simulink library "Wind_Lib"  (R2025a)
settings: Solver=ode45  StartTime=0.0  StopTime=10.0  RelTol=1e-3  EnableMultiTasking=on
undefined symbols (not defined in the file): WT_Params
libraries: nesl_utility x15, sm_lib x9, fl_lib x9, AerodynamicLoads_lib x1, $bdroot x1
Description:
  | Copyright 2009-2025 The MathWorks, Inc.
settings Model: Creator=smiller  LastModifiedBy=smiller
settings SolverCC: AlgebraicLoopSolver=TrustRegion
settings DataIOCC: LimitDataPoints=on  SaveFormat=Array  SignalLoggingSaveFormat=ModelDataLogs  ReturnWorkspaceOutputs=off
settings OptimizationCC: ReuseModelBlockBuffer=off  ExpressionDepthLimit=2147483647.0  LifeSpan=inf
settings DebuggingCC: UnderspecifiedInitializationDetection=Classic  MergeDetectMultiDrivingBlocksExec=none  SolverPrmCheckMsg=warning  FcnCallInpInsideContextMsg=warning  UnconnectedInputMsg=warning  UnconnectedOutputMsg=warning  UnconnectedLineMsg=warning  AllowSymbolicDim=off  StateNameClashWarn=warning  PregeneratedLibrarySubsystemCodeDiagnostic=none  SFUnexpectedBacktrackingDiag=warning  SFNoUnconditionalDefaultTransitionDiag=warning  SFExecutionAtInitializationDiag=none  ArithmeticOperatorsInVariantConditions=warning
settings HardwareCC: ProdBitPerPointer=32.0  ProdBitPerSizeT=32.0  ProdBitPerPtrDiffT=32.0  ProdLargestAtomicFloat=None  ProdIntDivRoundTo=Undefined  ProdEndianess=Unspecified  ProdWordSize=32.0  ProdHWDeviceType=32-bit Generic
settings ModelReferenceCC: EnableRefExpFcnMdlSchedulingChecks=on  PropagateSignalLabelsOutOfModel=off
settings SFSimCC: SimUseLocalCustomCode=off  CustomCodeUndefinedFunction=UseInterfaceOnly
settings RTWCC: RTWUseLocalCustomCode=off  GPUComputeCapability=3.5  DLArmComputeVersion=19.05
settings CodeAppCC: StateflowObjectComments=on
settings GRTTargetCC: TargetLangStandard=C89/C90 (ANSI)  CombineOutputUpdateFcns=off  GRTInterface=on
settings ConfigComp: CovMetricSettings=dw  CovSaveCumulativeToWorkspaceVar=on  CovSaveSingleToWorkspaceVar=on  CovExternalEMLEnable=off  CovSFcnEnable=off

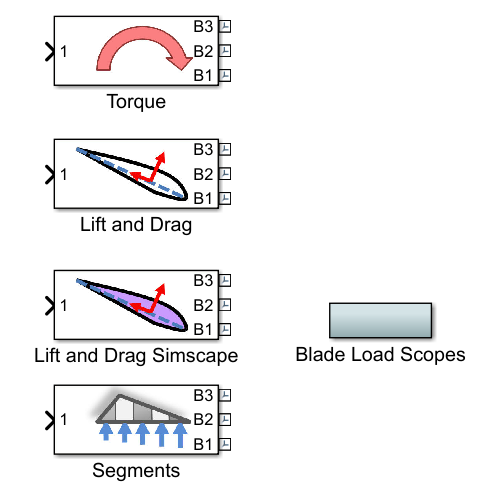
[thumbnail: Simulink's stored preview of the top-level diagram]
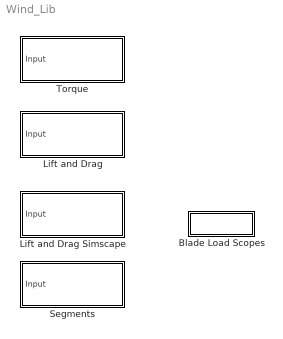
== system Wind_Lib ==
  Blade Load Scopes : Subsystem
  Lift and Drag : Subsystem
      mask Display: image('Blade_Load_Lift_Drag_IMAGE.jpg');
  Lift and Drag Simscape : Subsystem  VariantControl=Lift_and_Drag_Simscape
      mask Display: image('Blade_Load_Lift_Drag_SSC_IMAGE.jpg');
  Segments : Subsystem
      mask Display: image('Blade_Load_Segments_IMAGE.jpg');
  Torque : Subsystem
      mask Display: image('Blade_Load_Torque_IMAGE.jpg');

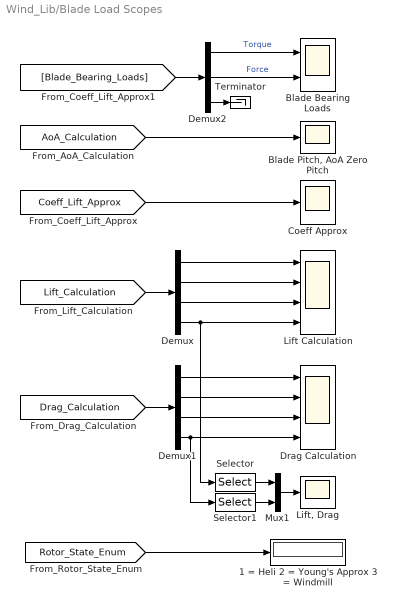
== system Wind_Lib/Blade Load Scopes ==
  1 = Heli 2 = Young's Approx 3 = Windmill : Display
  Blade Bearing Loads : Scope  NumInputPorts=2
      settings: TimeSpan=80  ActiveDisplayYMinimum=-2.0E+6  ActiveDisplayYMaximum=4.0E+6  DataLoggingVariableName=ScopeData10
  "Blade Pitch, AoA Zero Pitch" : Scope
      settings: TimeSpan=400  ActiveDisplayYMinimum=0  ActiveDisplayYMaximum=100  DataLoggingVariableName=ScopeData3
  Coeff Approx : Scope
      settings: TimeSpan=400  ActiveDisplayYMinimum=-0.1139986551164904  ActiveDisplayYMaximum=0.01794057021302797  DataLoggingVariableName=ScopeData4
  Demux : Demux  Outputs=[1 3 3 3]
  Demux1 : Demux  Outputs=[1 3 3 3]
  Demux2 : Demux  Outputs=[3 3 12]
  Drag Calculation : Scope  NumInputPorts=4
      settings: TimeSpan=400  ActiveDisplayYMinimum=-2000  ActiveDisplayYMaximum=4000  DataLoggingVariableName=ScopeData5
  Lift Calculation : Scope  NumInputPorts=4
      settings: TimeSpan=400  ActiveDisplayYMinimum=0  ActiveDisplayYMaximum=2000  DataLoggingVariableName=ScopeData2
  "Lift, Drag" : Scope
      settings: TimeSpan=160  ActiveDisplayYMinimum=-250.43517596694389  ActiveDisplayYMaximum=408.30262213523071
  Mux1 : Mux  Inputs=2
  Selector : Selector  InputPortWidth=3  IndexOptions=Index vector (dialog)  Indices=[1]  OutputSizes=1
  Selector1 : Selector  InputPortWidth=3  IndexOptions=Index vector (dialog)  Indices=[1 3]  OutputSizes=1
  Terminator : Terminator
  wires:
  Demux2/2 -> Blade Bearing Loads/2  "Force"
  Demux2/1 -> Blade Bearing Loads/1  "Torque"
  [Blade_Bearing_Loads] -> Demux2/1
  Selector1/1 -> Mux1/2
  Selector/1 -> Mux1/1
  [AoA_Calculation] -> "Blade Pitch, AoA Zero Pitch"/1
  Mux1/1 -> "Lift, Drag"/1
  [Lift_Calculation] -> Demux/1
  Demux/1 -> Lift Calculation/1
  Demux/2 -> Lift Calculation/2
  Demux/3 -> Lift Calculation/3
  Demux/4 -> Selector/1, Lift Calculation/4
  [Coeff_Lift_Approx] -> Coeff Approx/1
  [Drag_Calculation] -> Demux1/1
  Demux1/1 -> Drag Calculation/1
  Demux1/2 -> Drag Calculation/2
  Demux1/3 -> Drag Calculation/3
  Demux1/4 -> Selector1/1, Drag Calculation/4
  [Rotor_State_Enum] -> 1 = Heli 2 = Young's Approx 3 = Windmill/1
  Demux2/3 -> Terminator/1

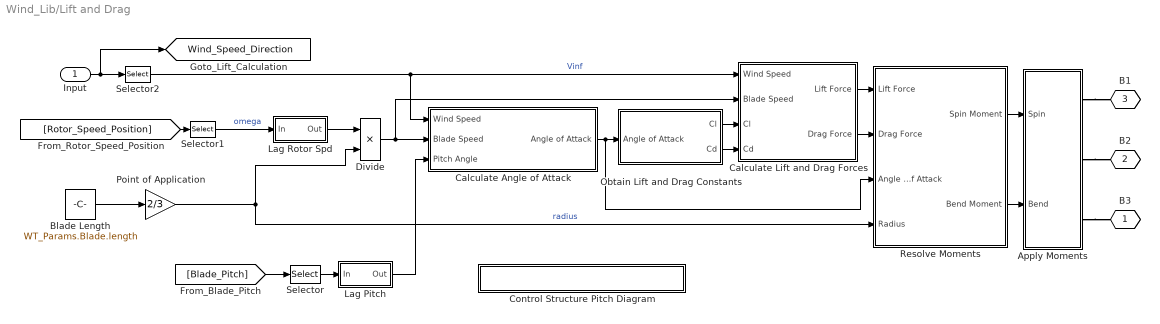
== system Wind_Lib/Lift and Drag ==
  Input : Inport
  Apply Moments : Subsystem
  Blade Length : Constant  Value=WT_Params.Blade.length
  Calculate Angle of Attack : Subsystem
  Calculate Lift and Drag Forces : Subsystem
  Control Structure Pitch Diagram : Subsystem
      mask Display: disp('View Blade Load Diagram');
  Divide : Product  Inputs=**
  Lag Pitch : Subsystem  mask(First-order lag supporting vector signals){b=WT_Params.Lift_Drag_Coeff.time_constant, x_initial=0}
      mask prompts: b "Filter time constant"; x_initial "Initial output"
      mask help: Models a lag of the form 1/(b*s+1) where s is the Laplace operator.
  Lag Rotor Spd : Subsystem  mask(First-order lag supporting vector signals){b=WT_Params.Lift_Drag_Coeff.time_constant, x_initial=0}
      mask prompts: b "Filter time constant"; x_initial "Initial output"
      mask help: Models a lag of the form 1/(b*s+1) where s is the Laplace operator.
  Obtain Lift and Drag Constants : Subsystem
  Point of Application : Gain  Gain=2/3
  Resolve Moments : Subsystem
  Selector : Selector  InputPortWidth=3  IndexOptions=Index vector (dialog)  Indices=[1]  OutputSizes=1
  Selector1 : Selector  InputPortWidth=2  IndexOptions=Index vector (dialog)  Indices=[2]  OutputSizes=1
  Selector2 : Selector  InputPortWidth=2  IndexOptions=Index vector (dialog)  Indices=[1]  OutputSizes=1
  B3 : PMIOPort  Tag=PMCPort  Side=Right
  B2 : PMIOPort  Tag=PMCPort  Port=2  Side=Right
  B1 : PMIOPort  Tag=PMCPort  Port=3  Side=Right
  tag scope: Wind_Speed_Direction=global
  wires:
  Selector/1 -> Lag Pitch/1(In)
  Lag Pitch/1(Out) -> Calculate Angle of Attack/3(Pitch Angle)
  Input/1 -> Selector2/1, [Wind_Speed_Direction]
  Selector2/1 -> Calculate Angle of Attack/1(Wind Speed), Calculate Lift and Drag Forces/1(Wind Speed)  "Vinf"
  Blade Length/1 -> Point of Application/1
  Divide/1 -> Calculate Angle of Attack/2(Blade Speed), Calculate Lift and Drag Forces/2(Blade Speed)
  [Blade_Pitch] -> Selector/1
  Calculate Angle of Attack/1(Angle of Attack) -> Obtain Lift and Drag Constants/1(Angle of Attack), Resolve Moments/3(Angle of Attack)
  Point of Application/1 -> Divide/2, Resolve Moments/4(Radius)  "radius"
  Resolve Moments/2(Bend Moment) -> Apply Moments/2(Bend)
  Resolve Moments/1(Spin Moment) -> Apply Moments/1(Spin)
  [Rotor_Speed_Position] -> Selector1/1
  Selector1/1 -> Lag Rotor Spd/1(In)  "omega"
  Obtain Lift and Drag Constants/1(Cl) -> Calculate Lift and Drag Forces/3(Cl)
  Obtain Lift and Drag Constants/2(Cd) -> Calculate Lift and Drag Forces/4(Cd)
  Calculate Lift and Drag Forces/1(Lift Force) -> Resolve Moments/1(Lift Force)
  Calculate Lift and Drag Forces/2(Drag Force) -> Resolve Moments/2(Drag Force)
  Lag Rotor Spd/1(Out) -> Divide/1
  connections:
  Apply Moments/RConn1 -- B1/RConn1
  Apply Moments/RConn2 -- B2/RConn1
  Apply Moments/RConn3 -- B3/RConn1

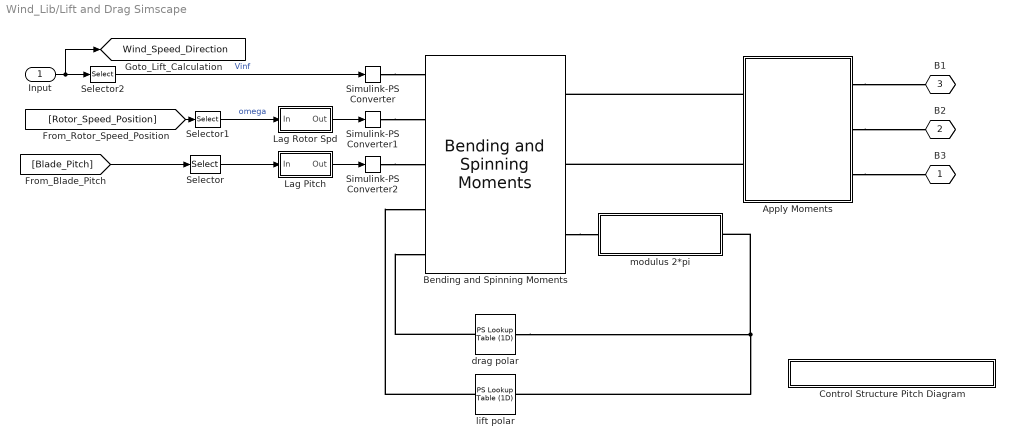
== system Wind_Lib/Lift and Drag Simscape ==
  Input : Inport
  Apply Moments : Subsystem
  Bending and Spinning Moments : AerodynamicLoads_lib/Bending and Spinning Moments  rho=WT_Params.Air.Density kg/m^3  blade_length=WT_Params.Blade.length m  blade_width=WT_Params.Blade.width m  ratio=0.66667  Fl_specify=off  Fl_priority=High  Fl=0 N  Fl_nominal_specify=off  Fl_nominal_value=1  Fl_nominal_unit=N  Fd_specify=off  Fd_priority=High  Fd=0 N  Fd_nominal_specify=off  Fd_nominal_value=1  Fd_nominal_unit=N  v_blade_specify=off  v_blade_priority=High  v_blade=0 m/s  v_blade_nominal_specify=off  v_blade_nominal_value=1  v_blade_nominal_unit=m/s  radius_specify=off  radius_priority=High  radius=0 m  radius_nominal_specify=off  radius_nominal_value=1  radius_nominal_unit=m
      settings: InternalSimscapePortConfiguration="{\"Bottom\":[],\"Left\":[{\"id\":\"v_wind\",\"label\":\"V_wind\",\"type\":\"input\"},{\"id\":\"w_rotor\",\"label\":\"w_rotor\",\"type\":\"input\"},{\"id\":\"theta\",\"label\":\"pitch_angle\",\"type\":\"input\"},{\"id\":\"Cl\",\"label\":\"CL\",\"type\":\"input\"},{\"id\":\"Cd\",\"label\":\"CD\",\"type\":\"input\"}],\"Right\":[{\"id\":\"spin_mom\",\"label\":\"spin\",\"type\":\"output\"},{\"id\":\"bend_mom\",\"label\":\"bend\",\"type\":\"output\"},{\"id\":\"AoA\",\"label\":\"AoA\",\"type\":\"output\"}],\"Top\":[]}"
  Control Structure Pitch Diagram : Subsystem
      mask Display: disp('View Blade Load Diagram');
  Lag Pitch : Subsystem  mask(First-order lag supporting vector signals){b=WT_Params.Lift_Drag_Coeff.time_constant, x_initial=0}
      mask prompts: b "Filter time constant"; x_initial "Initial output"
      mask help: Models a lag of the form 1/(b*s+1) where s is the Laplace operator.
  Lag Rotor Spd : Subsystem  mask(First-order lag supporting vector signals){b=WT_Params.Lift_Drag_Coeff.time_constant, x_initial=0}
      mask prompts: b "Filter time constant"; x_initial "Initial output"
      mask help: Models a lag of the form 1/(b*s+1) where s is the Laplace operator.
  Selector : Selector  InputPortWidth=3  IndexOptions=Index vector (dialog)  Indices=[1]  OutputSizes=1
  Selector1 : Selector  InputPortWidth=2  IndexOptions=Index vector (dialog)  Indices=[2]  OutputSizes=1
  Selector2 : Selector  InputPortWidth=2  IndexOptions=Index vector (dialog)  Indices=[1]  OutputSizes=1
  Simulink-PS Converter : nesl_utility/Simulink-PS Converter  PhysicalDomain=network_engine_domain  SubClassName=ps_input  LeftPortType=input  RightPortType=output  PseudoPeriodic=off  Frequencies=[]  NoiseDistribution=none  NoiseParameters=[]  Unit=m/s  AffineConversion=off  FilteringAndDerivatives=zero  SimscapeFilterOrder=1  InputFilterTimeConstant=0.005  UdotUserProvided=0
  Simulink-PS Converter1 : nesl_utility/Simulink-PS Converter  PhysicalDomain=network_engine_domain  SubClassName=ps_input  LeftPortType=input  RightPortType=output  PseudoPeriodic=off  Frequencies=[]  NoiseDistribution=none  NoiseParameters=[]  Unit=rad/s  AffineConversion=off  FilteringAndDerivatives=zero  SimscapeFilterOrder=1  InputFilterTimeConstant=0.005  UdotUserProvided=0
  Simulink-PS Converter2 : nesl_utility/Simulink-PS Converter  PhysicalDomain=network_engine_domain  SubClassName=ps_input  LeftPortType=input  RightPortType=output  PseudoPeriodic=off  Frequencies=[]  NoiseDistribution=none  NoiseParameters=[]  Unit=rad  AffineConversion=off  FilteringAndDerivatives=zero  SimscapeFilterOrder=1  InputFilterTimeConstant=0.005  UdotUserProvided=0
  drag polar : fl_lib/Physical Signals/Lookup Tables/PS Lookup Table (1D)  x=WT_Params.NACA0015.AoA  f=WT_Params.NACA0015.Cd  interp_method=1  extrap_method=1
  lift polar : fl_lib/Physical Signals/Lookup Tables/PS Lookup Table (1D)  x=WT_Params.NACA0015.AoA  f=WT_Params.NACA0015.Cl  interp_method=1  extrap_method=1
  modulus 2*pi : Subsystem
  B3 : PMIOPort  Tag=PMCPort  Side=Right
  B2 : PMIOPort  Tag=PMCPort  Port=2  Side=Right
  B1 : PMIOPort  Tag=PMCPort  Port=3  Side=Right
  tag scope: Wind_Speed_Direction=global
  wires:
  [Rotor_Speed_Position] -> Selector1/1
  [Blade_Pitch] -> Selector/1
  Input/1 -> [Wind_Speed_Direction], Selector2/1
  Selector2/1 -> Simulink-PS Converter/1  "Vinf"
  Selector1/1 -> Lag Rotor Spd/1(In)  "omega"
  Selector/1 -> Lag Pitch/1(In)
  Lag Rotor Spd/1(Out) -> Simulink-PS Converter1/1
  Lag Pitch/1(Out) -> Simulink-PS Converter2/1
  connections:
  Apply Moments/RConn3 -- B3/RConn1
  Apply Moments/RConn2 -- B2/RConn1
  Apply Moments/RConn1 -- B1/RConn1
  Simulink-PS Converter/RConn1 -- Bending and Spinning Moments/LConn1
  Simulink-PS Converter1/RConn1 -- Bending and Spinning Moments/LConn2
  Simulink-PS Converter2/RConn1 -- Bending and Spinning Moments/LConn3
  Bending and Spinning Moments/RConn3 -- modulus 2*pi/LConn1
  drag polar/LConn1 -- modulus 2*pi/RConn1 -- lift polar/LConn1
  drag polar/RConn1 -- Bending and Spinning Moments/LConn5
  lift polar/RConn1 -- Bending and Spinning Moments/LConn4
  Apply Moments/LConn1 -- Bending and Spinning Moments/RConn1
  Apply Moments/LConn2 -- Bending and Spinning Moments/RConn2

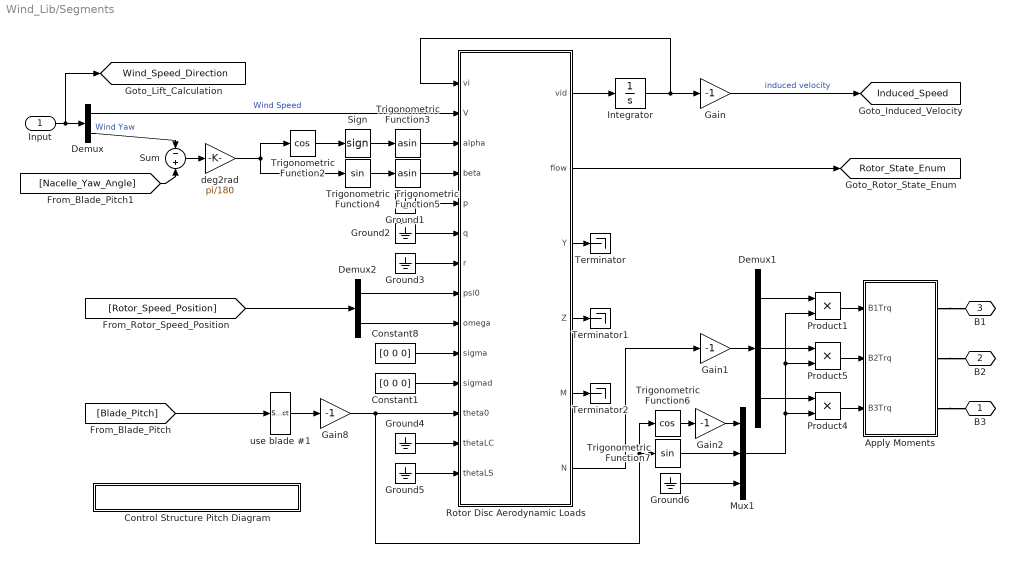
== system Wind_Lib/Segments ==
  Input : Inport
  Apply Moments : Subsystem
  Constant1 : Constant  Value=[0 0 0]
  Constant8 : Constant  Value=[0 0 0]
  Control Structure Pitch Diagram : Subsystem
      mask Display: disp('View Blade Load Diagram');
  Demux : Demux  Outputs=2
  Demux1 : Demux  Outputs=3
  Demux2 : Demux  Outputs=2
  Gain{,1..2,8} (4 alike) : Gain  Gain=-1
  Ground{1..6} (6 alike) : Ground
  Integrator : Integrator
  Mux1 : Mux  Inputs=3
  Product1 : Product  RndMeth=Zero
  Product4 : Product  RndMeth=Zero
  Product5 : Product  RndMeth=Zero
  Rotor Disc Aerodynamic Loads : MATLAB Function  TreatAsAtomicUnit=on  SystemSampleTime=0.01
  Sign : Signum
  Sum : Sum  Inputs=-|+
  Terminator : Terminator
  Terminator1 : Terminator
  Terminator2 : Terminator
  Trigonometric Function2 : Trigonometry  Operator=cos
  Trigonometric Function3 : Trigonometry  Operator=asin
  Trigonometric Function4 : Trigonometry
  Trigonometric Function5 : Trigonometry  Operator=asin
  Trigonometric Function6 : Trigonometry  Operator=cos
  Trigonometric Function7 : Trigonometry
  deg2rad : Gain  Gain=pi/180
  use blade #1 : Selector  InputPortWidth=3  IndexOptions=Index vector (dialog)  Indices=[1]  OutputSizes=1
  B3 : PMIOPort  Side=Right
  B2 : PMIOPort  Port=2  Side=Right
  B1 : PMIOPort  Port=3  Side=Right
  tag scope: Induced_Speed=global, Rotor_State_Enum=global, Wind_Speed_Direction=global
  wires:
  Rotor Disc Aerodynamic Loads/2(flow) -> [Rotor_State_Enum]
  [Rotor_Speed_Position] -> Demux2/1
  [Blade_Pitch] -> use blade #1/1
  Integrator/1 -> Gain/1, Rotor Disc Aerodynamic Loads/1(vi)
  Demux/1 -> Rotor Disc Aerodynamic Loads/2(V)  "Wind Speed"
  Demux/2 -> Sum/1  "Wind Yaw"
  Input/1 -> Demux/1, [Wind_Speed_Direction]
  Gain/1 -> [Induced_Speed]  "induced velocity"
  use blade #1/1 -> Gain8/1
  Gain8/1 -> Rotor Disc Aerodynamic Loads/12(theta0), Trigonometric Function7/1, Trigonometric Function6/1
  Ground1/1 -> Rotor Disc Aerodynamic Loads/5(p)
  Ground2/1 -> Rotor Disc Aerodynamic Loads/6(q)
  Ground3/1 -> Rotor Disc Aerodynamic Loads/7(r)
  Demux2/1 -> Rotor Disc Aerodynamic Loads/8(psi0)
  Demux2/2 -> Rotor Disc Aerodynamic Loads/9(omega)
  Constant8/1 -> Rotor Disc Aerodynamic Loads/10(sigma)
  Constant1/1 -> Rotor Disc Aerodynamic Loads/11(sigmad)
  Ground4/1 -> Rotor Disc Aerodynamic Loads/13(thetaLC)
  Ground5/1 -> Rotor Disc Aerodynamic Loads/14(thetaLS)
  Rotor Disc Aerodynamic Loads/1(vid) -> Integrator/1
  Rotor Disc Aerodynamic Loads/6(N) -> Gain1/1
  Rotor Disc Aerodynamic Loads/3(Y) -> Terminator/1
  Rotor Disc Aerodynamic Loads/4(Z) -> Terminator1/1
  Rotor Disc Aerodynamic Loads/5(M) -> Terminator2/1
  Trigonometric Function2/1 -> Sign/1
  Sign/1 -> Trigonometric Function3/1
  Trigonometric Function3/1 -> Rotor Disc Aerodynamic Loads/3(alpha)
  Trigonometric Function4/1 -> Trigonometric Function5/1
  Trigonometric Function5/1 -> Rotor Disc Aerodynamic Loads/4(beta)
  [Nacelle_Yaw_Angle] -> Sum/2
  Sum/1 -> deg2rad/1
  Ground6/1 -> Mux1/3
  Trigonometric Function7/1 -> Mux1/2
  Trigonometric Function6/1 -> Gain2/1
  Gain1/1 -> Demux1/1
  Demux1/1 -> Product1/1
  Demux1/2 -> Product5/1
  Demux1/3 -> Product4/1
  Mux1/1 -> Product4/2, Product1/2, Product5/2
  deg2rad/1 -> Trigonometric Function2/1, Trigonometric Function4/1
  Gain2/1 -> Mux1/1
  Product1/1 -> Apply Moments/1(B1Trq)
  Product5/1 -> Apply Moments/2(B2Trq)
  Product4/1 -> Apply Moments/3(B3Trq)
  connections:
  Apply Moments/RConn1 -- B1/RConn1
  Apply Moments/RConn2 -- B2/RConn1
  Apply Moments/RConn3 -- B3/RConn1

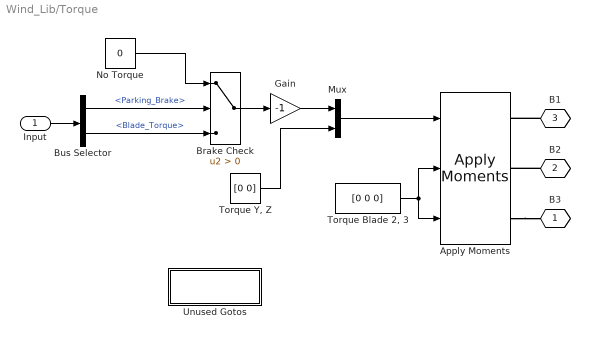
== system Wind_Lib/Torque ==
  Input : Inport
  Apply Moments : $bdroot/Segments/Apply Moments  SystemSampleTime=-1  VariantActivationTime=update diagram  EmptyChoice=off  PassThrough=off  PassThroughVariantControl=(default)  EmptyChoiceVariantControl=(default)  AllowFlexibleInterface=on  Latency=0  AutoFrameSizeCalculation=off
  Brake Check : Switch  Criteria=u2 > Threshold  SaturateOnIntegerOverflow=off  InputSameDT=off
  Bus Selector : BusSelector  OutputSignals=Parking_Brake,Blade_Torque
  Gain : Gain  Gain=-1
  Mux : Mux  Inputs=2
  No Torque : Constant  Value=0
  "Torque Blade 2, 3" : Constant  Value=[0 0 0]
  "Torque Y, Z" : Constant  Value=[0 0]
  Unused Gotos : Subsystem
  B3 : PMIOPort  Tag=PMCPort  Side=Right
  B2 : PMIOPort  Tag=PMCPort  Port=2  Side=Right
  B1 : PMIOPort  Tag=PMCPort  Port=3  Side=Right
  wires:
  Bus Selector/2 -> Brake Check/3  "<Blade_Torque>"
  Bus Selector/1 -> Brake Check/2  "<Parking_Brake>"
  No Torque/1 -> Brake Check/1
  "Torque Blade 2, 3"/1 -> Apply Moments/2, Apply Moments/3
  Mux/1 -> Apply Moments/1
  "Torque Y, Z"/1 -> Mux/2
  Input/1 -> Bus Selector/1
  Brake Check/1 -> Gain/1
  Gain/1 -> Mux/1
  connections:
  B1/RConn1 -- Apply Moments/RConn1
  B2/RConn1 -- Apply Moments/RConn2
  Apply Moments/RConn3 -- B3/RConn1

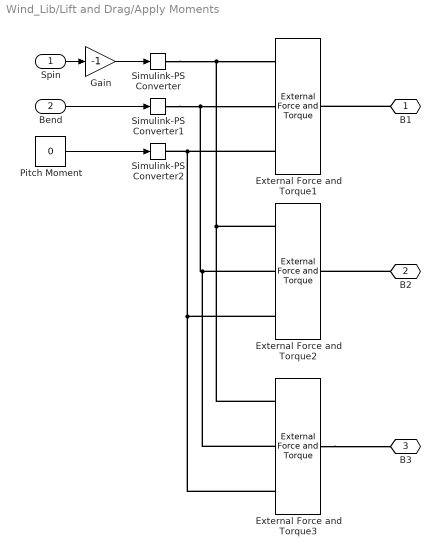
== system Wind_Lib/Lift and Drag/Apply Moments ==
  Spin : Inport
  Bend : Inport  Port=2
  External Force and Torque1 : sm_lib/Forces and Torques/External Force and Torque  EnableForceX=off  EnableForceY=off  EnableForceZ=off  EnableForce=off  ForceResolutionFrame=AttachedFrame  EnableTorqueX=on  EnableTorqueY=on  EnableTorqueZ=on  EnableTorque=off  TorqueResolutionFrame=AttachedFrame
  External Force and Torque2 : sm_lib/Forces and Torques/External Force and Torque  EnableForceX=off  EnableForceY=off  EnableForceZ=off  EnableForce=off  ForceResolutionFrame=AttachedFrame  EnableTorqueX=on  EnableTorqueY=on  EnableTorqueZ=on  EnableTorque=off  TorqueResolutionFrame=AttachedFrame
  External Force and Torque3 : sm_lib/Forces and Torques/External Force and Torque  EnableForceX=off  EnableForceY=off  EnableForceZ=off  EnableForce=off  ForceResolutionFrame=AttachedFrame  EnableTorqueX=on  EnableTorqueY=on  EnableTorqueZ=on  EnableTorque=off  TorqueResolutionFrame=AttachedFrame
  Gain : Gain  Gain=-1
  Pitch Moment : Constant  Value=0
  Simulink-PS Converter : nesl_utility/Simulink-PS Converter  PhysicalDomain=network_engine_domain  SubClassName=ps_input  LeftPortType=input  RightPortType=output  PseudoPeriodic=off  Frequencies=[]  NoiseDistribution=none  NoiseParameters=[]  Unit=1  AffineConversion=off  FilteringAndDerivatives=zero  SimscapeFilterOrder=1  InputFilterTimeConstant=0.005  UdotUserProvided=[]
  Simulink-PS Converter1 : nesl_utility/Simulink-PS Converter  PhysicalDomain=network_engine_domain  SubClassName=ps_input  LeftPortType=input  RightPortType=output  PseudoPeriodic=off  Frequencies=[]  NoiseDistribution=none  NoiseParameters=[]  Unit=1  AffineConversion=off  FilteringAndDerivatives=zero  SimscapeFilterOrder=1  InputFilterTimeConstant=0.005  UdotUserProvided=[]
  Simulink-PS Converter2 : nesl_utility/Simulink-PS Converter  PhysicalDomain=network_engine_domain  SubClassName=ps_input  LeftPortType=input  RightPortType=output  PseudoPeriodic=off  Frequencies=[]  NoiseDistribution=none  NoiseParameters=[]  Unit=1  AffineConversion=off  FilteringAndDerivatives=zero  SimscapeFilterOrder=1  InputFilterTimeConstant=0.005  UdotUserProvided=[]
  B1 : PMIOPort  Side=Right
  B2 : PMIOPort  Port=2  Side=Right
  B3 : PMIOPort  Port=3  Side=Right
  wires:
  Bend/1 -> Simulink-PS Converter1/1
  Gain/1 -> Simulink-PS Converter/1
  Pitch Moment/1 -> Simulink-PS Converter2/1
  Spin/1 -> Gain/1
  connections:
  Simulink-PS Converter/RConn1 -- External Force and Torque3/LConn1 -- External Force and Torque2/LConn1 -- External Force and Torque1/LConn1
  Simulink-PS Converter1/RConn1 -- External Force and Torque3/LConn2 -- External Force and Torque2/LConn2 -- External Force and Torque1/LConn2
  External Force and Torque1/LConn3 -- Simulink-PS Converter2/RConn1 -- External Force and Torque3/LConn3 -- External Force and Torque2/LConn3
  B1/RConn1 -- External Force and Torque1/RConn1
  B2/RConn1 -- External Force and Torque2/RConn1
  External Force and Torque3/RConn1 -- B3/RConn1

== system Wind_Lib/Lift and Drag/Calculate Angle of Attack ==
  Wind Speed : Inport
  Blade Speed : Inport  Port=2
  Pitch Angle : Inport  Port=3
  Subtract : Sum  Inputs=+-
  Trigonometric Function : Trigonometry  Operator=atan2
  Angle of Attack : Outport  VectorParamsAs1DForOutWhenUnconnected=off
  wires:
  Trigonometric Function/1 -> Subtract/1
  Wind Speed/1 -> Trigonometric Function/1
  Blade Speed/1 -> Trigonometric Function/2
  Subtract/1 -> Angle of Attack/1  "alpha"
  Pitch Angle/1 -> Subtract/2  "theta"

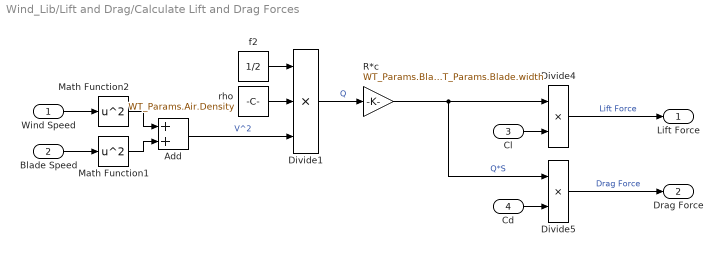
== system Wind_Lib/Lift and Drag/Calculate Lift and Drag Forces ==
  Wind Speed : Inport
  Blade Speed : Inport  Port=2
  Cl : Inport  Port=3
  Cd : Inport  Port=4
  Add : Sum
  Divide1 : Product  Inputs=***
  Divide4 : Product  Inputs=**
  Divide5 : Product  Inputs=**
  Math Function1 : Math  Operator=square  SignedPower=on
  Math Function2 : Math  Operator=square  SignedPower=on
  R*c : Gain  Gain=WT_Params.Blade.length*WT_Params.Blade.width
  f2 : Constant  Value=1/2
  rho : Constant  Value=WT_Params.Air.Density
  Lift Force : Outport  VectorParamsAs1DForOutWhenUnconnected=off
  Drag Force : Outport  Port=2  VectorParamsAs1DForOutWhenUnconnected=off
  wires:
  Math Function2/1 -> Add/1
  Math Function1/1 -> Add/2
  Add/1 -> Divide1/3  "V^2"
  rho/1 -> Divide1/2
  f2/1 -> Divide1/1
  Divide1/1 -> R*c/1  "Q"
  R*c/1 -> Divide4/1, Divide5/1  "Q*S"
  Wind Speed/1 -> Math Function2/1
  Blade Speed/1 -> Math Function1/1
  Divide4/1 -> Lift Force/1  "Lift Force"
  Cl/1 -> Divide4/2
  Divide5/1 -> Drag Force/1  "Drag Force"
  Cd/1 -> Divide5/2

== system Wind_Lib/Lift and Drag/Control Structure Pitch Diagram ==
  Subsystem : Subsystem
      mask Display: image(imread('Blade_Load_Calculation_IMAGE.jpg'));

== system Wind_Lib/Lift and Drag/Lag Pitch ==
  In : Inport
  Gain : Gain  Gain=1/b
  Integrator : Integrator  InitialCondition=x_initial
  Sum : Sum  Inputs=|+-  InputSameDT=on  SaturateOnIntegerOverflow=on  OutDataTypeStr=Inherit: Same as first input
  Out : Outport  VectorParamsAs1DForOutWhenUnconnected=off
  wires:
  Sum/1 -> Integrator/1
  In/1 -> Sum/1
  Integrator/1 -> Gain/1
  Gain/1 -> Sum/2, Out/1

== system Wind_Lib/Lift and Drag/Lag Rotor Spd ==
  In : Inport
  Gain : Gain  Gain=1/b
  Integrator : Integrator  InitialCondition=x_initial
  Sum : Sum  Inputs=|+-  InputSameDT=on  SaturateOnIntegerOverflow=on  OutDataTypeStr=Inherit: Same as first input
  Out : Outport  VectorParamsAs1DForOutWhenUnconnected=off
  wires:
  Gain/1 -> Out/1, Sum/2
  Integrator/1 -> Gain/1
  In/1 -> Sum/1
  Sum/1 -> Integrator/1

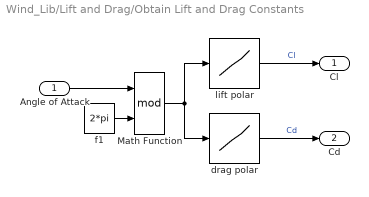
== system Wind_Lib/Lift and Drag/Obtain Lift and Drag Constants ==
  Angle of Attack : Inport
  Math Function : Math  Operator=mod  SignedPower=on
  drag polar : Lookup  InputValues=WT_Params.NACA0015.AoA  Table=WT_Params.NACA0015.Cd  SaturateOnIntegerOverflow=off
  f1 : Constant  Value=2*pi
  lift polar : Lookup  InputValues=WT_Params.NACA0015.AoA  Table=WT_Params.NACA0015.Cl  SaturateOnIntegerOverflow=off
  Cl : Outport  VectorParamsAs1DForOutWhenUnconnected=off
  Cd : Outport  Port=2  VectorParamsAs1DForOutWhenUnconnected=off
  wires:
  f1/1 -> Math Function/2
  Math Function/1 -> lift polar/1, drag polar/1
  Angle of Attack/1 -> Math Function/1
  lift polar/1 -> Cl/1  "Cl"
  drag polar/1 -> Cd/1  "Cd"

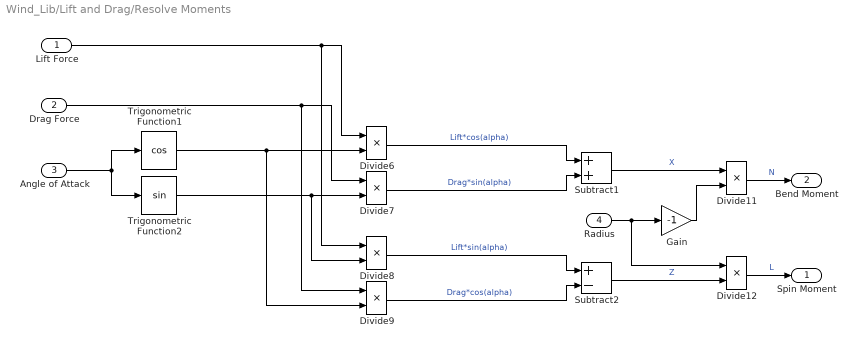
== system Wind_Lib/Lift and Drag/Resolve Moments ==
  Lift Force : Inport
  Drag Force : Inport  Port=2
  Angle of Attack : Inport  Port=3
  Radius : Inport  Port=4
  Divide{6..9,11..12} (6 alike) : Product  Inputs=**
  Gain : Gain  Gain=-1
  Subtract1 : Sum
  Subtract2 : Sum  Inputs=+-
  Trigonometric Function1 : Trigonometry  Operator=cos
  Trigonometric Function2 : Trigonometry
  Spin Moment : Outport  VectorParamsAs1DForOutWhenUnconnected=off
  Bend Moment : Outport  Port=2  VectorParamsAs1DForOutWhenUnconnected=off
  wires:
  Lift Force/1 -> Divide6/1, Divide8/1
  Drag Force/1 -> Divide7/1, Divide9/1
  Trigonometric Function1/1 -> Divide6/2, Divide9/2
  Trigonometric Function2/1 -> Divide7/2, Divide8/2
  Divide6/1 -> Subtract1/1  "Lift*cos(alpha)"
  Divide7/1 -> Subtract1/2  "Drag*sin(alpha)"
  Divide8/1 -> Subtract2/1  "Lift*sin(alpha)"
  Divide9/1 -> Subtract2/2  "Drag*cos(alpha)"
  Subtract1/1 -> Divide11/1  "X"
  Subtract2/1 -> Divide12/2  "Z"
  Gain/1 -> Divide11/2
  Angle of Attack/1 -> Trigonometric Function1/1, Trigonometric Function2/1
  Radius/1 -> Gain/1, Divide12/1
  Divide11/1 -> Bend Moment/1  "N"
  Divide12/1 -> Spin Moment/1  "L"

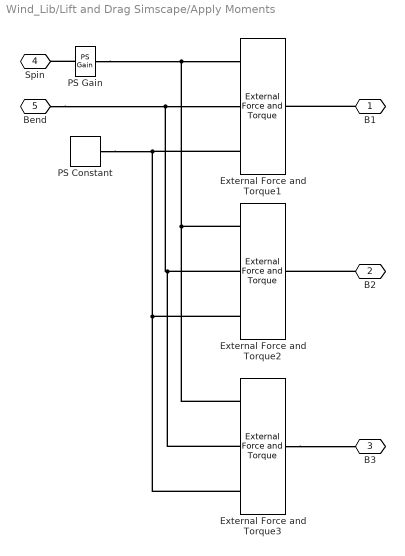
== system Wind_Lib/Lift and Drag Simscape/Apply Moments ==
  External Force and Torque1 : sm_lib/Forces and Torques/External Force and Torque  EnableForceX=off  EnableForceY=off  EnableForceZ=off  EnableForce=off  ForceResolutionFrame=AttachedFrame  EnableTorqueX=on  EnableTorqueY=on  EnableTorqueZ=on  EnableTorque=off  TorqueResolutionFrame=AttachedFrame
  External Force and Torque2 : sm_lib/Forces and Torques/External Force and Torque  EnableForceX=off  EnableForceY=off  EnableForceZ=off  EnableForce=off  ForceResolutionFrame=AttachedFrame  EnableTorqueX=on  EnableTorqueY=on  EnableTorqueZ=on  EnableTorque=off  TorqueResolutionFrame=AttachedFrame
  External Force and Torque3 : sm_lib/Forces and Torques/External Force and Torque  EnableForceX=off  EnableForceY=off  EnableForceZ=off  EnableForce=off  ForceResolutionFrame=AttachedFrame  EnableTorqueX=on  EnableTorqueY=on  EnableTorqueZ=on  EnableTorque=off  TorqueResolutionFrame=AttachedFrame
  PS Constant : fl_lib/Physical Signals/Sources/PS Constant  constant=0
  PS Gain : fl_lib/Physical Signals/Functions/PS Gain  gain=-1
  B1 : PMIOPort  Side=Right
  B2 : PMIOPort  Port=2  Side=Right
  B3 : PMIOPort  Port=3  Side=Right
  Spin : PMIOPort  Port=4  Side=Left
  Bend : PMIOPort  Port=5  Side=Left
  connections:
  External Force and Torque3/LConn1 -- External Force and Torque2/LConn1 -- PS Gain/RConn1 -- External Force and Torque1/LConn1
  External Force and Torque3/LConn2 -- External Force and Torque2/LConn2 -- Bend/RConn1 -- External Force and Torque1/LConn2
  External Force and Torque1/LConn3 -- PS Constant/RConn1 -- External Force and Torque3/LConn3 -- External Force and Torque2/LConn3
  B1/RConn1 -- External Force and Torque1/RConn1
  B2/RConn1 -- External Force and Torque2/RConn1
  External Force and Torque3/RConn1 -- B3/RConn1
  PS Gain/LConn1 -- Spin/RConn1

== system Wind_Lib/Lift and Drag Simscape/Control Structure Pitch Diagram ==
  Subsystem : Subsystem
      mask Display: image(imread('Blade_Load_Calculation_IMAGE.jpg'));

== system Wind_Lib/Lift and Drag Simscape/Lag Pitch ==
  In : Inport
  Gain : Gain  Gain=1/b
  Integrator : Integrator  InitialCondition=x_initial
  Sum : Sum  Inputs=|+-  InputSameDT=on  SaturateOnIntegerOverflow=on  OutDataTypeStr=Inherit: Same as first input
  Out : Outport  VectorParamsAs1DForOutWhenUnconnected=off
  wires:
  Sum/1 -> Integrator/1
  In/1 -> Sum/1
  Integrator/1 -> Gain/1
  Gain/1 -> Sum/2, Out/1

== system Wind_Lib/Lift and Drag Simscape/Lag Rotor Spd ==
  In : Inport
  Gain : Gain  Gain=1/b
  Integrator : Integrator  InitialCondition=x_initial
  Sum : Sum  Inputs=|+-  InputSameDT=on  SaturateOnIntegerOverflow=on  OutDataTypeStr=Inherit: Same as first input
  Out : Outport  VectorParamsAs1DForOutWhenUnconnected=off
  wires:
  Gain/1 -> Out/1, Sum/2
  Integrator/1 -> Gain/1
  In/1 -> Sum/1
  Sum/1 -> Integrator/1

== system Wind_Lib/Lift and Drag Simscape/modulus 2*pi ==
  2*pi : fl_lib/Physical Signals/Sources/PS Constant  constant=2*pi rad
  PS Divide : fl_lib/Physical Signals/Functions/PS Divide
  PS Floor : fl_lib/Physical Signals/Nonlinear Operators/PS Floor
      settings: InternalSimscapePortConfiguration="{\"Bottom\":[],\"Left\":[{\"id\":\"I\",\"label\":\"\",\"type\":\"input\"}],\"Right\":[{\"id\":\"O\",\"label\":\"\",\"type\":\"output\"}],\"Top\":[]}"
  PS Product : fl_lib/Physical Signals/Functions/PS Product
  PS Subtract : fl_lib/Physical Signals/Functions/PS Subtract
  AoA : PMIOPort  Side=Left
  mod(AoA,2*pi) : PMIOPort  Port=2  Side=Right
  connections:
  2*pi/RConn1 -- PS Product/LConn2 -- PS Divide/LConn2
  AoA/RConn1 -- PS Subtract/LConn1 -- PS Divide/LConn1
  PS Divide/RConn1 -- PS Floor/LConn1
  PS Product/LConn1 -- PS Floor/RConn1
  PS Subtract/LConn2 -- PS Product/RConn1
  mod(AoA,2*pi)/RConn1 -- PS Subtract/RConn1

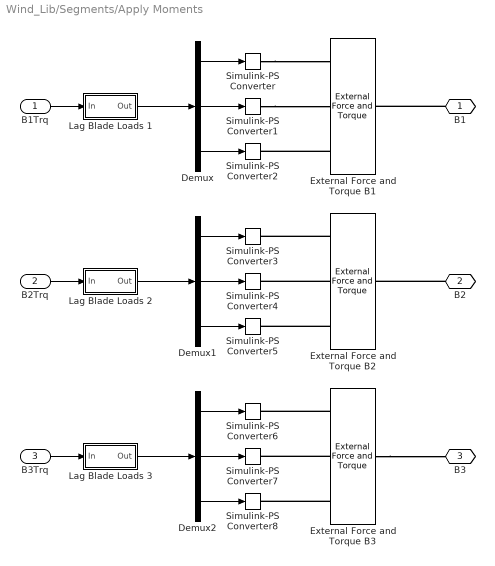
== system Wind_Lib/Segments/Apply Moments ==
  B1Trq : Inport
  B2Trq : Inport  Port=2
  B3Trq : Inport  Port=3
  Demux : Demux  Outputs=3
  Demux1 : Demux  Outputs=3
  Demux2 : Demux  Outputs=3
  External Force and Torque B1 : sm_lib/Forces and Torques/External Force and Torque  EnableForceX=off  EnableForceY=off  EnableForceZ=off  EnableForce=off  ForceResolutionFrame=AttachedFrame  EnableTorqueX=on  EnableTorqueY=on  EnableTorqueZ=on  EnableTorque=off  TorqueResolutionFrame=AttachedFrame
  External Force and Torque B3 : sm_lib/Forces and Torques/External Force and Torque  EnableForceX=off  EnableForceY=off  EnableForceZ=off  EnableForce=off  ForceResolutionFrame=AttachedFrame  EnableTorqueX=on  EnableTorqueY=on  EnableTorqueZ=on  EnableTorque=off  TorqueResolutionFrame=AttachedFrame
  External Force and Torque B2 : sm_lib/Forces and Torques/External Force and Torque  EnableForceX=off  EnableForceY=off  EnableForceZ=off  EnableForce=off  ForceResolutionFrame=AttachedFrame  EnableTorqueX=on  EnableTorqueY=on  EnableTorqueZ=on  EnableTorque=off  TorqueResolutionFrame=AttachedFrame
  Lag Blade Loads 1 : Subsystem  mask(First-order lag supporting vector signals){b=WT_Params.Lift_Drag_Coeff.time_constant, x_initial=0}
      mask prompts: b "Filter time constant"; x_initial "Initial output"
      mask help: Models a lag of the form 1/(b*s+1) where s is the Laplace operator.
  Lag Blade Loads 2 : Subsystem  mask(First-order lag supporting vector signals){b=WT_Params.Lift_Drag_Coeff.time_constant, x_initial=0}
      mask prompts: b "Filter time constant"; x_initial "Initial output"
      mask help: Models a lag of the form 1/(b*s+1) where s is the Laplace operator.
  Lag Blade Loads 3 : Subsystem  mask(First-order lag supporting vector signals){b=WT_Params.Lift_Drag_Coeff.time_constant, x_initial=0}
      mask prompts: b "Filter time constant"; x_initial "Initial output"
      mask help: Models a lag of the form 1/(b*s+1) where s is the Laplace operator.
  Simulink-PS Converter{,1..8} (9 alike) : nesl_utility/Simulink-PS Converter  PhysicalDomain=network_engine_domain  SubClassName=ps_input  LeftPortType=input  RightPortType=output  PseudoPeriodic=off  Frequencies=[]  NoiseDistribution=none  NoiseParameters=[]  Unit=1  AffineConversion=off  FilteringAndDerivatives=zero  SimscapeFilterOrder=1  InputFilterTimeConstant=0.005  UdotUserProvided=[]
  B1 : PMIOPort  Side=Right
  B2 : PMIOPort  Port=2  Side=Right
  B3 : PMIOPort  Port=3  Side=Right
  wires:
  B1Trq/1 -> Lag Blade Loads 1/1(In)
  Demux/1 -> Simulink-PS Converter/1
  Demux/2 -> Simulink-PS Converter1/1
  Demux/3 -> Simulink-PS Converter2/1
  B2Trq/1 -> Lag Blade Loads 2/1(In)
  Demux1/1 -> Simulink-PS Converter3/1
  Demux1/2 -> Simulink-PS Converter4/1
  Demux1/3 -> Simulink-PS Converter5/1
  B3Trq/1 -> Lag Blade Loads 3/1(In)
  Demux2/1 -> Simulink-PS Converter6/1
  Demux2/2 -> Simulink-PS Converter7/1
  Demux2/3 -> Simulink-PS Converter8/1
  Lag Blade Loads 1/1(Out) -> Demux/1
  Lag Blade Loads 2/1(Out) -> Demux1/1
  Lag Blade Loads 3/1(Out) -> Demux2/1
  connections:
  Simulink-PS Converter/RConn1 -- External Force and Torque B1/LConn1
  Simulink-PS Converter1/RConn1 -- External Force and Torque B1/LConn2
  External Force and Torque B1/LConn3 -- Simulink-PS Converter2/RConn1
  B1/RConn1 -- External Force and Torque B1/RConn1
  B2/RConn1 -- External Force and Torque B2/RConn1
  External Force and Torque B3/RConn1 -- B3/RConn1
  External Force and Torque B2/LConn3 -- Simulink-PS Converter5/RConn1
  External Force and Torque B2/LConn2 -- Simulink-PS Converter4/RConn1
  External Force and Torque B2/LConn1 -- Simulink-PS Converter3/RConn1
  External Force and Torque B3/LConn1 -- Simulink-PS Converter6/RConn1
  External Force and Torque B3/LConn3 -- Simulink-PS Converter8/RConn1
  External Force and Torque B3/LConn2 -- Simulink-PS Converter7/RConn1

== system Wind_Lib/Segments/Control Structure Pitch Diagram ==
  Subsystem : Subsystem
      mask Display: image(imread('Blade_Load_Calculation_IMAGE.jpg'));

== system Wind_Lib/Torque/Unused Gotos ==
  Constant : Constant  Value=0
  Constant2 : Constant  Value=zeros(1,10)
  tag scope: AoA_Calculation=global, Coeff_Lift_Approx=global, Drag_Calculation=global, Lift_Calculation=global
  wires:
  Constant2/1 -> [Drag_Calculation], [Lift_Calculation]
  Constant/1 -> [Coeff_Lift_Approx], [AoA_Calculation]

== system Wind_Lib/Lift and Drag/Control Structure Pitch Diagram/Subsystem ==

== system Wind_Lib/Lift and Drag Simscape/Control Structure Pitch Diagram/Subsystem ==

== system Wind_Lib/Segments/Apply Moments/Lag Blade Loads 1 ==
  In : Inport
  Gain : Gain  Gain=1/b
  Integrator : Integrator  InitialCondition=x_initial
  Sum : Sum  Inputs=|+-  InputSameDT=on  SaturateOnIntegerOverflow=on  OutDataTypeStr=Inherit: Same as first input
  Out : Outport  VectorParamsAs1DForOutWhenUnconnected=off
  wires:
  Sum/1 -> Integrator/1
  In/1 -> Sum/1
  Integrator/1 -> Gain/1
  Gain/1 -> Sum/2, Out/1

== system Wind_Lib/Segments/Apply Moments/Lag Blade Loads 2 ==
  In : Inport
  Gain : Gain  Gain=1/b
  Integrator : Integrator  InitialCondition=x_initial
  Sum : Sum  Inputs=|+-  InputSameDT=on  SaturateOnIntegerOverflow=on  OutDataTypeStr=Inherit: Same as first input
  Out : Outport  VectorParamsAs1DForOutWhenUnconnected=off
  wires:
  Gain/1 -> Out/1, Sum/2
  Integrator/1 -> Gain/1
  In/1 -> Sum/1
  Sum/1 -> Integrator/1

== system Wind_Lib/Segments/Apply Moments/Lag Blade Loads 3 ==
  In : Inport
  Gain : Gain  Gain=1/b
  Integrator : Integrator  InitialCondition=x_initial
  Sum : Sum  Inputs=|+-  InputSameDT=on  SaturateOnIntegerOverflow=on  OutDataTypeStr=Inherit: Same as first input
  Out : Outport  VectorParamsAs1DForOutWhenUnconnected=off
  wires:
  Sum/1 -> Integrator/1
  In/1 -> Sum/1
  Integrator/1 -> Gain/1
  Gain/1 -> Sum/2, Out/1

== system Wind_Lib/Segments/Control Structure Pitch Diagram/Subsystem ==

== matlab function Wind_Lib/Segments/Rotor Disc Aerodynamic Loads ==
  data Y settings: description=blade force y components [N] (in disc plane)
  data Z settings: description=blade force z components [N] (perpendicular disc plane)
  data M settings: description=blade moment y component [Nm] (flapping)
  data N settings: description=blade moment z component [Nm] (shaft torque)
  data: vi input size=1; V input size=1; alpha input size=1; beta input size=1; p input size=1; q input size=1; r input size=1; psi0 input size=1; omega input size=1; sigma input; sigmad input; theta0 input size=1; thetaLC input size=1; thetaLS input size=1; WT_Params parameter; vid output size=1; flow output size=1; Y output; Z output; M output; N output

function [...
    vid,  ... induced velocity rate    [m/s^2]
    flow, ... rotor state: 1:heli 2:young 3:windmill
    Y,    ... blade force y components [N]  (in disc plane)
    Z,    ... blade force z components [N]  (perpendicular disc plane)
    M,    ... blade moment y component [Nm] (flapping)
    N     ... blade moment z component [Nm] (shaft torque)
    ] ...
    = Rotor( ...
... states
    vi,       ... induced velocity       [m/s]
    V,        ... airspeed freestream    [m/s] [0..inf[
    alpha,    ... disc angle-of-attack   [rad]
    beta,     ... disc angle-of-sideslip [rad]
    p,        ... disc rate-of-rotation  [rad/s] (about principal axis)
    q,        ...
    r,        ...
    psi0,     ... blade #0 azimuth       [rad]
    omega,    ... shaft angular rate     [rad/s]
    sigma,    ... blade flap angles      [rad]
    sigmad,   ... blade flap angle rates [rad/s]
... controls
    theta0,   ... collective pitch command          [rad]
    thetaLC,  ... longitudinal cyclic pitch command [rad]
    thetaLS,  ... lateral cyclic pitch command      [rad]
... parameters
    WT_Params ...
)

persistent psi I s J
persistent R c AR CLmax CLa CD0 k CDmax
persistent rho a
persistent ds


if isempty(I)

    % blades
    psi = zeros(1,length(sigma));
    I = length(psi);  % number of blades (evenly spaced)

    % spanwise segmentation
    s = zeros(10,1);  % CHANGE HERE
    J = length(s);     % number of spanwise segments


    % rotor
    R     = WT_Params.Blade.length;  % rotor radius  [m]
    c     = WT_Params.Blade.width;   % blade choord  [m]
    AR    = R^2/(c*R);               % blade aspect ratio (approximation)
    CLmax = WT_Params.Rotor.MaxLiftCoefficent;        % max(min) lift coefficient
    CLa   = 2*pi /( 1 + 2/AR );                       % lift coefficient gradient
    CD0   = WT_Params.Rotor.ParasiteDragCoefficient;  % parasite drag coefficient
    k     = WT_Params.Rotor.InducedDragFactor;        % induced drag factor
    CDmax = WT_Params.Rotor.MaxDragCoefficient;       % max drag coefficient

    % atmosphere
    rho   = WT_Params.Air.Density;       % air density    [kg/m^3]
    a     = WT_Params.Air.SpeedOfSound;  % speed of sound [m/s]


    % blade relative angles
    for i = 1 : I,  psi(i) = 2*pi *(i-1)/I;  end

    % spanwise segment length and position
    ds = R /J;
    for j = 1 : J,  s(j) = ds/2 + (j-1) *ds;  end

end


% airspeed components and angle-of-incidence
v = V            *sin( beta );
u = (V^2-v^2)^.5 *cos( alpha );
w = (V^2-v^2)^.5 *sin( alpha );
if u==0 && v==0,
    if w >= 0, gamma = -pi/2;
    else       gamma = +pi/2;
    end
else           gamma = atan( -w/(u*u+v*v)^.5 );
end


% Agenda
%
%  1 calc. Thrust at current Induced Velocity using Blade Element Theory (BET)
%  2 calc. Thrust at current Induced Velocity using Linear Momentum Theory (LMT)
%  3 calc. Induced Velocity rate of change


% Thrust at current Induced Velocity using Blade Element Theory (BET)
Y = zeros(length(psi),1);
Z = zeros(length(psi),1);
M = zeros(length(psi),1);
N = zeros(length(psi),1);

for i = 1 : I  % parse all blades

    cos_psi = cos( psi0 + psi(i) );
    sin_psi = sin( psi0 + psi(i) );

    % blade pitch angle
    theta = theta0 + thetaLC *cos_psi + thetaLS *sin_psi;

    for j = 1 : J  % parse all spanwise segments

        % blade spanwise total airspeed
        UT = u *sin_psi + v *cos_psi + s(j) *( omega + sigma(i) *( p *cos_psi - q *sin_psi ) - r );
        UP = w - sigma(i) *( u *cos_psi - v *sin_psi ) - vi + s(j) *( - sigmad(i) + p *sin_psi + q *cos_psi );
        U2  = ( UT^2 + UP^2 );
        U  = U2^.5;

        % blade spanwise inflow angle, [-180..+180] deg
        phi = atan2( UP, UT );
        cos_phi = cos( phi );
        sin_phi = sin( phi );

        % blade spanwise apparent angle-of-attack, [0..180] deg
        AoA = mod( theta + phi, pi );

        % blade spanwise mach number (clamped) and wave drag factor
        mach = U /a;
        if 0.9 < mach
            mach = 0.9;
        end
        WD = 1 /( 1 - mach^2 );

        % blade spanwise angle-of-attack @ stall
        AoAstall = CLmax /( WD *CLa );
        if AoAstall <= 0 || AoAstall > pi/2
            AoAstall = pi/2;
        end

        % blade spanwise aerodynamic coefficients
        if AoA <= AoAstall,           % interval [0..AoAstall]
            CL = CLa *AoA;
            CD = WD *CD0 + k *CL^2;
            CL = WD *CL;
        elseif AoA >= pi - AoAstall,  % interval [pi-AoAstall..pi]
            CL = CLa *( AoA - pi );
            CD = WD *CD0 + k *CL^2;
            CL = WD *CL;
        else                          % interval [AoAstall..pi-AoAstall]
            delta = ( AoA - pi/2 ) /( AoAstall - pi/2 );
            CL = CLmax *delta;
            CD = CDmax + ( WD *CD0 + k *( CLmax /WD )^2 - CDmax ) *delta^2;
        end

        % blade spanwise dynamic pressure, lift and drag forces
        Q = .5 *rho *U2 *c *ds;
        dLift = Q *CL;
        dDrag = Q *CD;

        % blade segment forces and moments
        dY = - dLift *sin_phi + dDrag *cos_phi;
        dZ = - dLift *cos_phi - dDrag *sin_phi;
        dM = - s(j) *dZ;
        dN =   s(j) *dY;

        % total blade force and moment
        Y(i) = Y(i) + dY;
        Z(i) = Z(i) + dZ;
        M(i) = M(i) + dM;
        N(i) = N(i) + dN;

    end

end

TBET = - sum( Z );


% Thrust at current Induced Velocity using Linear Momentum Theory (LMT)

if gamma >= 0,  % climb and hover

    % flow is reversed when vi < -V/2

    % when flow is not reversed, use derived formula
    if -V/2 <= vi
        TLMT = 2*rho*pi*R^2*vi*( (V*cos(gamma))^2+(V*sin(gamma)+vi)^2 )^.5;
        flow = 1;
    else

        % when flow is reversed, use approximation by Young
        A = ( (5-4*sin(gamma))^.5 - 5^.5 ) /( 1-5^.5 );
        if -5/3*V < vi
            TLMT = 2*rho*pi*R^2*( -A*((vi-3*V)/7)^2 + (1-A)*vi*(V^2+vi^2)^.5 );
            flow = 2;
        else
            TLMT = 2*rho*pi*R^2*( -A*(vi+V)^2       + (1-A)*vi*(V^2+vi^2)^.5 );
            flow = 3;
        end

    end

else  % descent,  (gamma < 0)

    % flow is reversed when vi > V/2

    % when flow is not reversed, use derived formula
    if V/2 >= vi
        TLMT = 2*rho*pi*R^2*vi*( (V*cos(gamma))^2+(-V*sin(gamma)-vi)^2 )^.5;
        flow = 1;
    else

        % when flow is reversed, use approximation by Young
        A = ( (5+4*sin(gamma))^.5 - 5^.5 ) /( 1-5^.5 );
        if 5/3*V > vi
            TLMT = 2*rho*pi*R^2*( A*((vi+3*V)/7)^2 + (1-A)*vi*(V^2+vi^2)^.5 );
            flow = 2;
        else
            TLMT = 2*rho*pi*R^2*( A*( vi-V     )^2 + (1-A)*vi*(V^2+vi^2)^.5 );
            flow = 3;
        end

    end

end


% Induced Velocity rate of change

h = R;
vid = ( TBET - TLMT ) /rho /pi /R^2 /h;



% TODO
%eml.extrinsic('myread');


% -- eof
